simulink model "ex1"  (R2025b)
settings: Solver=FixedStepAuto  StartTime=0.0  StopTime=0.16  FixedStep=1e-5  RelTol=1e-4
values from neighbouring files (symbols this model uses):
  In = 20    [sim1.m]
  J = 0.001    [sim1.m]
  L = 2.5e-3    (= 0.0025)    [sim1.m]
  psi = 0.35    [sim1.m]
  R = 0.5    [sim1.m]
  Tn = 7    [sim1.m]
  Vn = 120    [sim1.m]
  wn = Nn*2*pi/60    (= 314.159265359)    [sim1.m]
settings Model: Creator=dimit  LastModifiedBy=Dimitris

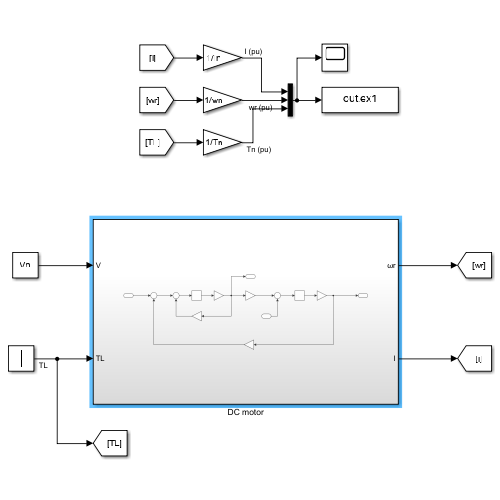
[thumbnail: Simulink's stored preview of the top-level diagram]
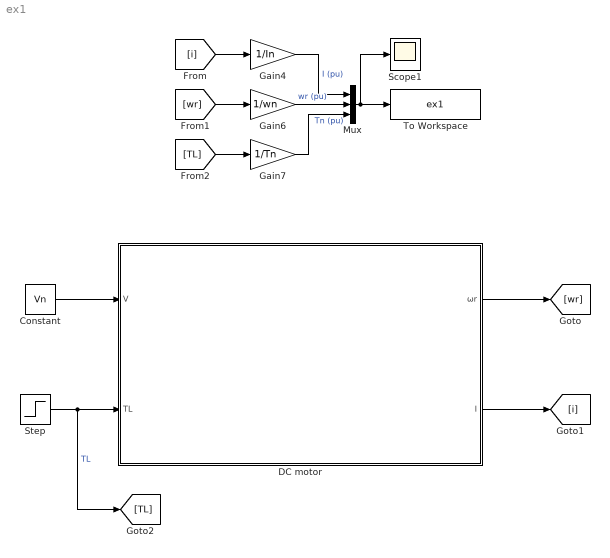
== system ex1 ==
  Constant : Constant  Value=Vn
  DC motor : Subsystem
  Gain4 : Gain  Gain=1/In
  Gain6 : Gain  Gain=1/wn
  Gain7 : Gain  Gain=1/Tn
  Mux : Mux  Inputs=3
  Scope1 : Scope
      settings: ActiveDisplayYMinimum=-2.1980660085413319  ActiveDisplayYMaximum=7.1388671048691359
  Step : Step  Time=0.1  After=Tn  SampleTime=0
  To Workspace : ToWorkspace  VariableName=ex1  SaveFormat=Timeseries  SampleTime=-1
  wires:
  [i] -> Gain4/1
  [wr] -> Gain6/1
  Gain6/1 -> Mux/2  "wr (pu)"
  Gain4/1 -> Mux/1  "I (pu)"
  Mux/1 -> Scope1/1, To Workspace/1
  [TL] -> Gain7/1
  Gain7/1 -> Mux/3  "Tn (pu)"
  Constant/1 -> DC motor/1(V)
  DC motor/1(ωr) -> [wr]
  DC motor/2(I) -> [i]
  Step/1 -> [TL], DC motor/2(TL)  "TL"

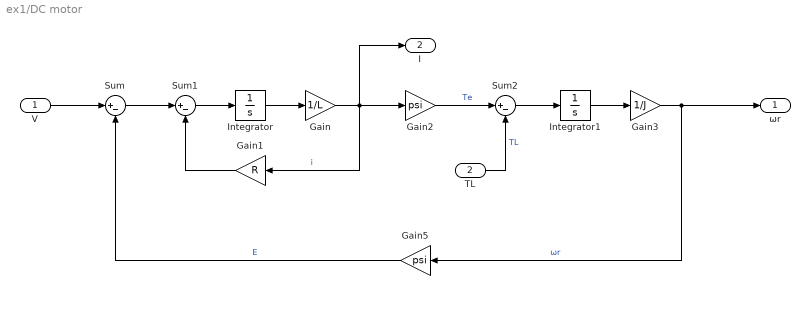
== system ex1/DC motor ==
  V : Inport
  TL : Inport  Port=2
  Gain : Gain  Gain=1/L
  Gain1 : Gain  Gain=R
  Gain2 : Gain  Gain=psi
  Gain3 : Gain  Gain=1/J
  Gain5 : Gain  Gain=psi
  Integrator : Integrator
  Integrator1 : Integrator
  Sum : Sum  Inputs=|+-
  Sum1 : Sum  Inputs=|+-
  Sum2 : Sum  Inputs=|+-
  ωr : Outport
  I : Outport  Port=2
  wires:
  Gain3/1 -> ωr/1, Gain5/1  "ωr"
  Integrator/1 -> Gain/1
  Sum1/1 -> Integrator/1
  Gain2/1 -> Sum2/1  "Te"
  TL/1 -> Sum2/2  "TL"
  Sum/1 -> Sum1/1
  Gain1/1 -> Sum1/2
  Integrator1/1 -> Gain3/1
  Sum2/1 -> Integrator1/1
  Gain/1 -> I/1, Gain2/1, Gain1/1  "i"
  Gain5/1 -> Sum/2  "E"
  V/1 -> Sum/1
